simulink model "motor_arduino_simulink"  (R2023b)
settings: Solver=FixedStepDiscrete  StartTime=0.0  StopTime=inf  FixedStep=0.01  RelTol=1e-3  EnableMultiTasking=on
InitFcn:
  | PPR = 7;
  | Ts = 0.01;
  | GR = 300;
libraries: slpidlib x2, arduinolib x2, arduinosensorlib x1, simulink x1
settings Model: ExtModeTrigDuration=2  Creator=ManJit  LastModifiedBy=ManJit
settings SolverCC: AutoInsertRateTranBlk=on
settings OptimizationCC: EnhancedBackFolding=on  PassReuseOutputArgsAs=Individual arguments  ZeroExternalMemoryAtStartup=off  ZeroInternalMemoryAtStartup=off  MaxStackSize=64  OptimizeBlockOrder=speed  DifferentSizesBufferReuse=on  OptimizationCustomize=off  EfficientTunableParamExpr=on
settings DebuggingCC: ParameterTunabilityLossMsg=error
settings HardwareCC: ProdBitPerInt=16  ProdBitPerPointer=16  ProdBitPerSizeT=16  ProdBitPerPtrDiffT=16  ProdLargestAtomicInteger=Integer  ProdLargestAtomicFloat=None  ProdWordSize=8  ProdHWDeviceType=Atmel->AVR
settings SFSimCC: MATLABDynamicMemAlloc=off
settings RTWCC: Description=Embedded Coder  SystemTargetFile=ert.tlc  HardwareBoard=Arduino Nano 3.0  TemplateMakefile=ert_default_tmf  Toolchain=Arduino AVR  BuildConfiguration=Faster Runs
settings CodeAppCC: ForceParamTrailComments=on  IgnoreCustomStorageClasses=off  OperatorAnnotations=on  SimulinkDataObjDesc=on  SFDataObjDesc=on  InsertBlockDesc=on
settings ERTTargetCC: SupportContinuousTime=on  SupportVariableSizeSignals=on  ExtModeTransport=3  ExtModeStaticAlloc=on  ExtModeAutomaticAllocSize=off  ExtModeStaticAllocSize=250  ExtModeMexFile=ext_xcp  ExtModeIntrfLevel=Level2 - Open

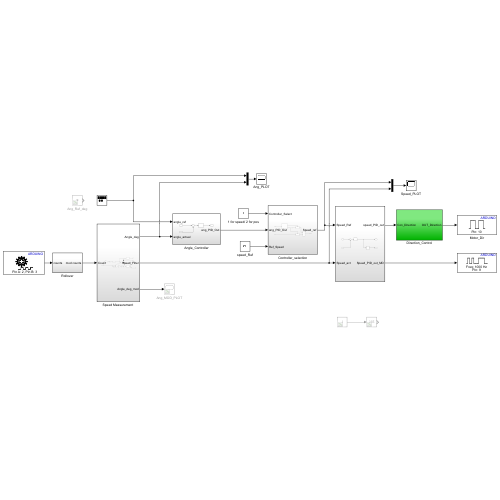
[thumbnail: Simulink's stored preview of the top-level diagram]
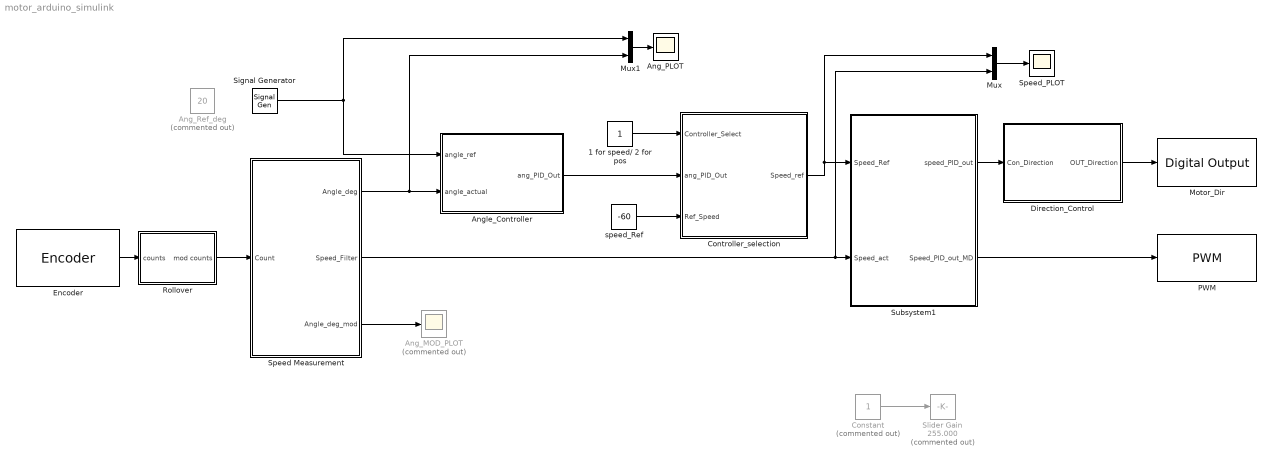
== system motor_arduino_simulink ==
  1 for speed/ 2 for pos : Constant
  Ang_MOD_PLOT : Scope  Commented=on
  Ang_PLOT : Scope
  Ang_Ref_deg : Constant  Commented=on  Value=20
  Angle_Controller : Subsystem
  Constant : Constant  Commented=on
  Controller_selection : Subsystem
  Direction_Control : Subsystem
  Encoder : arduinosensorlib/Encoder  InputA=2  InputB=3  Mode=No reset  SampleTime=-1
  Motor_Dir : arduinolib/Digital Output  pinNumber=10  Direction=output  blockPlatform=arduino
  Mux : Mux  Inputs=2
  Mux1 : Mux  Inputs=2
  PWM : arduinolib/PWM  pinNumber=9  frequencyType=Specify  desiredFrequency=1000  achievableFrequency=1000
  Rollover : Subsystem
  Signal Generator : SignalGenerator  Amplitude=100  Frequency=0.1
  Slider Gain : simulink/Math Operations/Slider Gain  Commented=on  gain=255.000  low=0  high=255
  "Speed Measurement " : Subsystem
  Speed_PLOT : Scope
  Subsystem1 : Subsystem
  speed_Ref : Constant  Value=-60
  wires:
  Encoder/1 -> Rollover/1(counts)
  Constant/1 -> Slider Gain/1
  Rollover/1(" mod counts") -> "Speed Measurement "/1(Count)
  Direction_Control/1(OUT_Direction) -> Motor_Dir/1
  "Speed Measurement "/2(Speed_Filter) -> Mux/2, Subsystem1/2(Speed_act)
  Subsystem1/1(speed_PID_out) -> Direction_Control/1(Con_Direction)
  Subsystem1/2(Speed_PID_out_MD) -> PWM/1
  1 for speed/ 2 for pos/1 -> Controller_selection/1(Controller_Select)
  Angle_Controller/1(ang_PID_Out) -> Controller_selection/2(ang_PID_Out)
  Controller_selection/1(Speed_ref) -> Mux/1, Subsystem1/1(Speed_Ref)
  speed_Ref/1 -> Controller_selection/3(Ref_Speed)
  Mux/1 -> Speed_PLOT/1
  Mux1/1 -> Ang_PLOT/1
  "Speed Measurement "/3(Angle_deg_mod) -> Ang_MOD_PLOT/1
  "Speed Measurement "/1(Angle_deg) -> Mux1/2, Angle_Controller/2(angle_actual)
  Signal Generator/1 -> Angle_Controller/1(angle_ref), Mux1/1

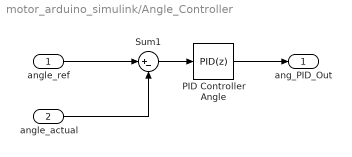
== system motor_arduino_simulink/Angle_Controller ==
  angle_ref : Inport
  angle_actual : Inport  Port=2
  PID Controller Angle : slpidlib/PID Controller  Controller=PID  Form=Parallel  TimeDomain=Discrete-time  UseExternalTs=off  SampleTime=0.02  IntegratorMethod=Forward Euler  FilterMethod=Forward Euler  ControllerParametersSource=internal  P=1  I=0.05  UseKiTs=off  D=0  N=10  UseFilter=on  TunerSelectOption=Transfer Function Based (PID Tuner App)  InitialConditionSource=internal  InitialConditionForIntegrator=0  InitialConditionForFilter=0  DifferentiatorICPrevScaledInput=0  ExternalReset=none  TrackingMode=off  Kt=1  LimitOutput=on  SatLimitsSource=internal  UpperSaturationLimit=60  LowerSaturationLimit=-60  LinearizeAsGain=on  AntiWindupMode=clamping  Kb=1  LimitIntegrator=off  UpperIntegratorSaturationLimit=inf  LowerIntegratorSaturationLimit=-inf  POutMin=[]  POutMax=[]  IOutMin=[]  IOutMax=[]  DOutMin=[]  DOutMax=[]  NOutMin=[]  NOutMax=[]  SumOutMin=[]  SumOutMax=[]  SaturationOutMin=[]  SaturationOutMax=[]  PParamMin=[]  PParamMax=[]  IParamMin=[]  IParamMax=[]  DParamMin=[]  DParamMax=[]  NParamMin=[]  NParamMax=[]  KbParamMin=[]  KbParamMax=[]  KtParamMin=[]  KtParamMax=[]  KbOutMin=[]  KbOutMax=[]  KtOutMin=[]  KtOutMax=[]  IntegratorOutMin=[]  IntegratorOutMax=[]  FilterOutMin=[]  FilterOutMax=[]  SumI1OutMin=[]  SumI1OutMax=[]  SumI2OutMin=[]  SumI2OutMax=[]  SumI3OutMin=[]  SumI3OutMax=[]  SumI4OutMin=[]  SumI4OutMax=[]  SumDOutMin=[]  SumDOutMax=[]  DifferentiatorOutMin=[]  DifferentiatorOutMax=[]  FilterDiffOutCoefMin=[]  FilterDiffOutCoefMax=[]  ReciprocalOutMin=[]  ReciprocalOutMax=[]  SumDenOutMin=[]  SumDenOutMax=[]  SumNumOutMin=[]  SumNumOutMax=[]  DivideOutMin=[]  DivideOutMax=[]  UdiffTsProdOutMin=[]  UdiffTsProdOutMax=[]  NTsProdOutMin=[]  NTsProdOutMax=[]  UintegralTsProdOutMin=[]  UintegralTsProdOutMax=[]  UngainTsProdOutMin=[]  UngainTsProdOutMax=[]  ClampingZeroOutDataTypeStr=Inherit: Inherit via back propagation  ClampingZeroOutMin=[]  ClampingZeroOutMax=[]  FilterDenConstantOutDataTypeStr=Inherit: Inherit via back propagation  FilterDenConstantOutMin=[]  FilterDenConstantOutMax=[]  PCopyOutDataTypeStr=Inherit: Inherit via back propagation  PCopyOutMin=[]  PCopyOutMax=[]  NCopyOutDataTypeStr=Inherit: Inherit via back propagation  NCopyOutMin=[]  NCopyOutMax=[]  IntegratorContinuousStateAttributes=''  IntegratorStateMustResolveToSignalObject=off  IntegratorRTWStateStorageClass=Auto  FilterContinuousStateAttributes=''  FilterStateMustResolveToSignalObject=off  FilterRTWStateStorageClass=Auto  ParallelPVariant=InternalParameters  IdealPVariant=Disabled  IVariant=InternalParameters  DVariant=InternalParameters  IntegratorVariant=Discrete  SatVariant=Enabled  AWVariant=DiscClampingParallel  PCopyVariant=Disabled  TRVariant=Disabled  FdbkBlocksVariant=Forward  IdealPFdbkVariant=Disabled  SatFdbkVariant=Disabled  DerivativeFilterVariant=ForwardEulerFilter  NVariant=InternalParameters  NCopyVariant=Disabled  FilterICVariant=InternalICsFilter  IntegratorICVariant=InternalICs  ExternalResetVariant=Disabled  TRSumVariant=Passthrough  SumFdbkVariant=Disabled  SumVariant=Sum_PID  TsampFilterVariant=InternalTs  TsampNgainVariant=Passthrough  TsampIntegralVariant=Disabled_SignalSpec  ExternalSaturationOutDataTypeStr=Inherit: Same as second input
  Sum1 : Sum  Inputs=|+-
  ang_PID_Out : Outport
  wires:
  PID Controller Angle/1 -> ang_PID_Out/1
  Sum1/1 -> PID Controller Angle/1
  angle_actual/1 -> Sum1/2
  angle_ref/1 -> Sum1/1

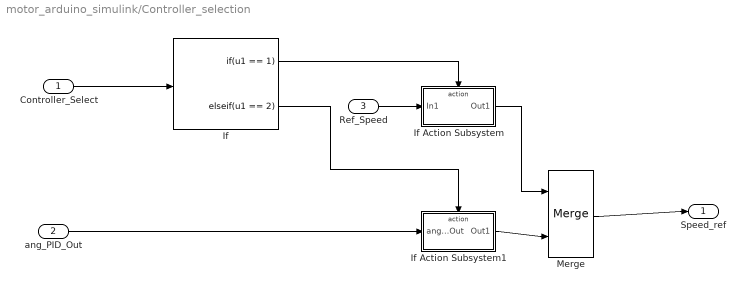
== system motor_arduino_simulink/Controller_selection ==
  Controller_Select : Inport
  ang_PID_Out : Inport  Port=2
  Ref_Speed : Inport  Port=3
  If : If  IfExpression=u1 == 1  ElseIfExpressions=u1 == 2  ShowElse=off
  If Action Subsystem : Subsystem  TreatAsAtomicUnit=on
  If Action Subsystem1 : Subsystem  TreatAsAtomicUnit=on
  Merge : Merge
  Speed_ref : Outport
  wires:
  Controller_Select/1 -> If/1
  ang_PID_Out/1 -> If Action Subsystem1/1(ang_PID_Out)
  If Action Subsystem/1(Out1) -> Merge/1
  If/1 -> If Action Subsystem/Action
  If/2 -> If Action Subsystem1/Action
  If Action Subsystem1/1(Out1) -> Merge/2
  Merge/1 -> Speed_ref/1
  Ref_Speed/1 -> If Action Subsystem/1(In1)

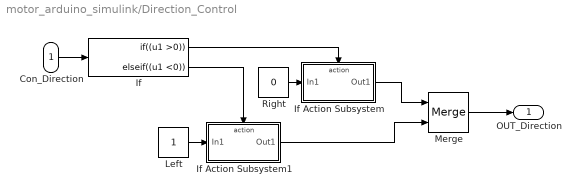
== system motor_arduino_simulink/Direction_Control ==
  Con_Direction : Inport
  If : If  IfExpression=(u1 >0)  ElseIfExpressions=(u1 <0)  ShowElse=off
  If Action Subsystem : Subsystem  TreatAsAtomicUnit=on
  If Action Subsystem1 : Subsystem  TreatAsAtomicUnit=on
  Left : Constant
  Merge : Merge
  Right : Constant  Value=0
  OUT_Direction : Outport  VectorParamsAs1DForOutWhenUnconnected=off
  wires:
  If Action Subsystem1/1(Out1) -> Merge/2
  If/1 -> If Action Subsystem/Action
  If Action Subsystem/1(Out1) -> Merge/1
  Con_Direction/1 -> If/1
  Right/1 -> If Action Subsystem/1(In1)
  Left/1 -> If Action Subsystem1/1(In1)
  If/2 -> If Action Subsystem1/Action
  Merge/1 -> OUT_Direction/1

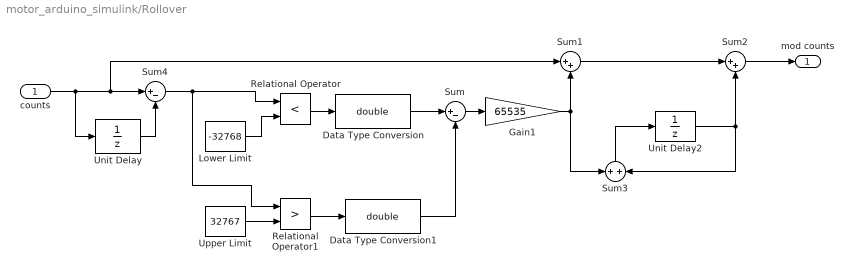
== system motor_arduino_simulink/Rollover ==
  counts : Inport
  " Lower Limit" : Constant  Value=-32768
  " Upper Limit" : Constant  Value=32767
  Data Type Conversion : DataTypeConversion  OutDataTypeStr=double  SaturateOnIntegerOverflow=off
  Data Type Conversion1 : DataTypeConversion  OutDataTypeStr=double  SaturateOnIntegerOverflow=off
  Gain1 : Gain  Gain=65535
  Relational Operator : RelationalOperator  Operator=<  OutDataTypeStr=boolean  InputSameDT=off
  Relational Operator1 : RelationalOperator  Operator=>  OutDataTypeStr=boolean  InputSameDT=off
  Sum : Sum  Inputs=|+-
  Sum1 : Sum  Inputs=|++
  Sum2 : Sum  Inputs=|++
  Sum3 : Sum
  Sum4 : Sum  Inputs=|+-
  Unit Delay : UnitDelay  SampleTime=-1  HasFrameUpgradeWarning=on
  Unit Delay2 : UnitDelay  SampleTime=-1  HasFrameUpgradeWarning=on
  " mod counts" : Outport
  wires:
  counts/1 -> Unit Delay/1, Sum1/1, Sum4/1
  Sum2/1 -> " mod counts"/1
  Unit Delay/1 -> Sum4/2
  Data Type Conversion/1 -> Sum/1
  Sum3/1 -> Unit Delay2/1
  Data Type Conversion1/1 -> Sum/2
  Sum/1 -> Gain1/1
  Gain1/1 -> Sum1/2, Sum3/1
  Relational Operator1/1 -> Data Type Conversion1/1
  Sum1/1 -> Sum2/1
  Relational Operator/1 -> Data Type Conversion/1
  " Upper Limit"/1 -> Relational Operator1/2
  Unit Delay2/1 -> Sum3/2, Sum2/2
  " Lower Limit"/1 -> Relational Operator/2
  Sum4/1 -> Relational Operator/1, Relational Operator1/1

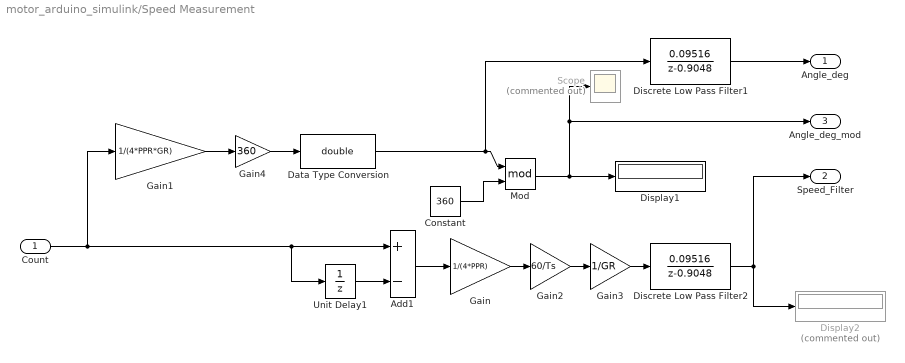
== system motor_arduino_simulink/Speed Measurement  ==
  Count : Inport
  Add1 : Sum  Inputs=+-
  Constant : Constant  Value=360
  Data Type Conversion : DataTypeConversion  OutDataTypeStr=double  SaturateOnIntegerOverflow=off  RndMeth=Floor
  Discrete Low Pass Filter1 : DiscreteTransferFcn  Numerator=[0.09516]  Denominator=[1 -0.9048]
  Discrete Low Pass Filter2 : DiscreteTransferFcn  Numerator=[0.09516]  Denominator=[1 -0.9048]
  Display1 : Display
  Display2 : Display  Commented=on
  Gain : Gain  Gain=1/(4*PPR)
  Gain1 : Gain  Gain=1/(4*PPR*GR)
  Gain2 : Gain  Gain=60/Ts
  Gain3 : Gain  Gain=1/GR
  Gain4 : Gain  Gain=360
  Mod : Math  Operator=mod
  Scope : Scope  Commented=on
  Unit Delay1 : UnitDelay  SampleTime=-1  HasFrameUpgradeWarning=on
  Angle_deg : Outport
  Speed_Filter : Outport  Port=2
  Angle_deg_mod : Outport  Port=3
  wires:
  Gain/1 -> Gain2/1
  Unit Delay1/1 -> Add1/2
  Count/1 -> Add1/1, Unit Delay1/1, Gain1/1
  Discrete Low Pass Filter2/1 -> Speed_Filter/1, Display2/1
  Gain2/1 -> Gain3/1
  Add1/1 -> Gain/1
  Gain3/1 -> Discrete Low Pass Filter2/1
  Gain4/1 -> Data Type Conversion/1
  Constant/1 -> Mod/2
  Mod/1 -> Display1/1, Scope/1, Angle_deg_mod/1
  Gain1/1 -> Gain4/1
  Data Type Conversion/1 -> Discrete Low Pass Filter1/1, Mod/1
  Discrete Low Pass Filter1/1 -> Angle_deg/1

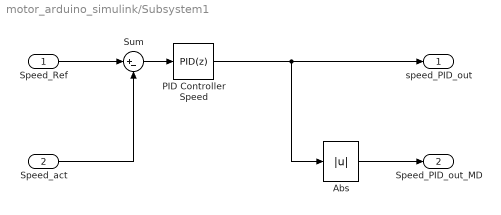
== system motor_arduino_simulink/Subsystem1 ==
  Speed_Ref : Inport
  Speed_act : Inport  Port=2
  Abs : Abs  SaturateOnIntegerOverflow=off
  PID Controller Speed : slpidlib/PID Controller  Controller=PID  Form=Parallel  TimeDomain=Discrete-time  UseExternalTs=off  SampleTime=0.01  IntegratorMethod=Forward Euler  FilterMethod=Forward Euler  ControllerParametersSource=internal  P=25  I=30  UseKiTs=off  D=0.1  N=100  UseFilter=on  TunerSelectOption=Transfer Function Based (PID Tuner App)  InitialConditionSource=internal  InitialConditionForIntegrator=0  InitialConditionForFilter=0  DifferentiatorICPrevScaledInput=0  ExternalReset=none  TrackingMode=off  Kt=1  LimitOutput=on  SatLimitsSource=internal  UpperSaturationLimit=255  LowerSaturationLimit=-255  LinearizeAsGain=on  AntiWindupMode=clamping  Kb=1  LimitIntegrator=off  UpperIntegratorSaturationLimit=inf  LowerIntegratorSaturationLimit=-inf  POutMin=[]  POutMax=[]  IOutMin=[]  IOutMax=[]  DOutMin=[]  DOutMax=[]  NOutMin=[]  NOutMax=[]  SumOutMin=[]  SumOutMax=[]  SaturationOutMin=[]  SaturationOutMax=[]  PParamMin=[]  PParamMax=[]  IParamMin=[]  IParamMax=[]  DParamMin=[]  DParamMax=[]  NParamMin=[]  NParamMax=[]  KbParamMin=[]  KbParamMax=[]  KtParamMin=[]  KtParamMax=[]  KbOutMin=[]  KbOutMax=[]  KtOutMin=[]  KtOutMax=[]  IntegratorOutMin=[]  IntegratorOutMax=[]  FilterOutMin=[]  FilterOutMax=[]  SumI1OutMin=[]  SumI1OutMax=[]  SumI2OutMin=[]  SumI2OutMax=[]  SumI3OutMin=[]  SumI3OutMax=[]  SumI4OutMin=[]  SumI4OutMax=[]  SumDOutMin=[]  SumDOutMax=[]  DifferentiatorOutMin=[]  DifferentiatorOutMax=[]  FilterDiffOutCoefMin=[]  FilterDiffOutCoefMax=[]  ReciprocalOutMin=[]  ReciprocalOutMax=[]  SumDenOutMin=[]  SumDenOutMax=[]  SumNumOutMin=[]  SumNumOutMax=[]  DivideOutMin=[]  DivideOutMax=[]  UdiffTsProdOutMin=[]  UdiffTsProdOutMax=[]  NTsProdOutMin=[]  NTsProdOutMax=[]  UintegralTsProdOutMin=[]  UintegralTsProdOutMax=[]  UngainTsProdOutMin=[]  UngainTsProdOutMax=[]  ClampingZeroOutDataTypeStr=Inherit: Inherit via back propagation  ClampingZeroOutMin=[]  ClampingZeroOutMax=[]  FilterDenConstantOutDataTypeStr=Inherit: Inherit via back propagation  FilterDenConstantOutMin=[]  FilterDenConstantOutMax=[]  PCopyOutDataTypeStr=Inherit: Inherit via back propagation  PCopyOutMin=[]  PCopyOutMax=[]  NCopyOutDataTypeStr=Inherit: Inherit via back propagation  NCopyOutMin=[]  NCopyOutMax=[]  IntegratorContinuousStateAttributes=''  IntegratorStateMustResolveToSignalObject=off  IntegratorRTWStateStorageClass=Auto  FilterContinuousStateAttributes=''  FilterStateMustResolveToSignalObject=off  FilterRTWStateStorageClass=Auto  ParallelPVariant=InternalParameters  IdealPVariant=Disabled  IVariant=InternalParameters  DVariant=InternalParameters  IntegratorVariant=Discrete  SatVariant=Enabled  AWVariant=DiscClampingParallel  PCopyVariant=Disabled  TRVariant=Disabled  FdbkBlocksVariant=Forward  IdealPFdbkVariant=Disabled  SatFdbkVariant=Disabled  DerivativeFilterVariant=ForwardEulerFilter  NVariant=InternalParameters  NCopyVariant=Disabled  FilterICVariant=InternalICsFilter  IntegratorICVariant=InternalICs  ExternalResetVariant=Disabled  TRSumVariant=Passthrough  SumFdbkVariant=Disabled  SumVariant=Sum_PID  TsampFilterVariant=InternalTs  TsampNgainVariant=Passthrough  TsampIntegralVariant=Disabled_SignalSpec  ExternalSaturationOutDataTypeStr=Inherit: Same as second input
  Sum : Sum  Inputs=|+-
  speed_PID_out : Outport
  Speed_PID_out_MD : Outport  Port=2
  wires:
  Speed_Ref/1 -> Sum/1
  PID Controller Speed/1 -> Abs/1, speed_PID_out/1
  Sum/1 -> PID Controller Speed/1
  Speed_act/1 -> Sum/2
  Abs/1 -> Speed_PID_out_MD/1

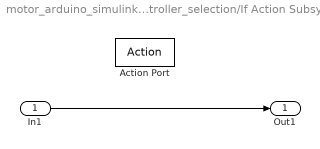
== system motor_arduino_simulink/Controller_selection/If Action Subsystem ==
  In1 : Inport
  Action Port : ActionPort  ActionPortLabel=if(u1 == 1)
  Out1 : Outport
  wires:
  In1/1 -> Out1/1

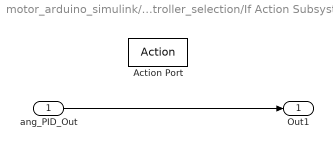
== system motor_arduino_simulink/Controller_selection/If Action Subsystem1 ==
  ang_PID_Out : Inport
  Action Port : ActionPort  ActionPortLabel=elseif(u1 == 2)
  Out1 : Outport  VectorParamsAs1DForOutWhenUnconnected=off
  wires:
  ang_PID_Out/1 -> Out1/1

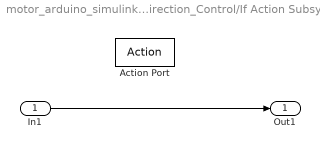
== system motor_arduino_simulink/Direction_Control/If Action Subsystem ==
  In1 : Inport
  Action Port : ActionPort  ActionPortLabel=if((u1 >0))
  Out1 : Outport  VectorParamsAs1DForOutWhenUnconnected=off
  wires:
  In1/1 -> Out1/1

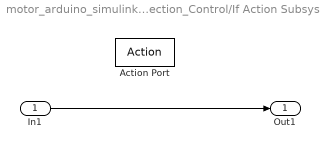
== system motor_arduino_simulink/Direction_Control/If Action Subsystem1 ==
  In1 : Inport
  Action Port : ActionPort  ActionPortLabel=elseif((u1 <0))
  Out1 : Outport  VectorParamsAs1DForOutWhenUnconnected=off
  wires:
  In1/1 -> Out1/1
